simulink model "Trench_Zone"  (R2023b)
settings: Solver=VariableStepAuto  StartTime=0.0  StopTime=10.0  RelTol=1e-3
undefined symbols (not defined in the file or in its folder): Need_Distance_from_Trench, Warning_Threshold_Max_Distance, Warning_Threshold_Min_Distance, Warning_Threshold_Time
settings Model: Creator=Bing  LastModifiedBy=Bing

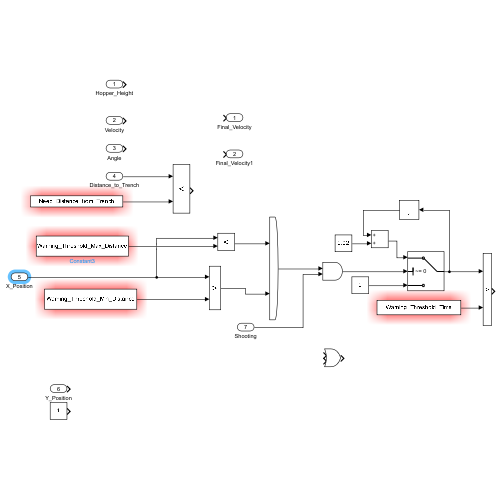
[thumbnail: Simulink's stored preview of the top-level diagram]
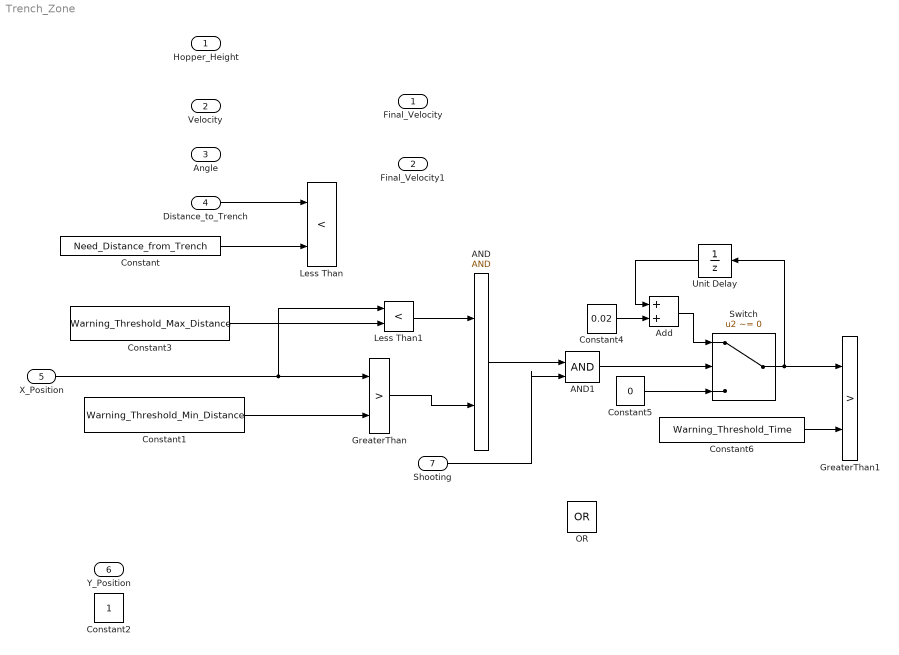
== system Trench_Zone ==
  Hopper_Height : Inport
  Velocity : Inport  Port=2
  Angle : Inport  Port=3
  Distance_to_Trench : Inport  Port=4
  X_Position : Inport  Port=5
  Y_Position : Inport  Port=6
  Shooting : Inport  Port=7
  AND : Logic  IconShape=distinctive  AllPortsSameDT=off  OutDataTypeStr=boolean
  AND1 : Logic  IconShape=distinctive  AllPortsSameDT=off  OutDataTypeStr=boolean
  Add : Sum
  Constant : Constant  Value=Need_Distance_from_Trench
  Constant1 : Constant  Value=Warning_Threshold_Min_Distance
  Constant2 : Constant
  Constant3 : Constant  Value=Warning_Threshold_Max_Distance
  Constant4 : Constant  Value=0.02
  Constant5 : Constant  Value=0
  Constant6 : Constant  Value=Warning_Threshold_Time
  GreaterThan : RelationalOperator  Operator=>  OutDataTypeStr=boolean  RndMeth=Simplest  InputSameDT=off
  GreaterThan1 : RelationalOperator  Operator=>  OutDataTypeStr=boolean  RndMeth=Simplest  InputSameDT=off
  Less Than : RelationalOperator  Operator=<  OutDataTypeStr=boolean  RndMeth=Simplest  InputSameDT=off
  Less Than1 : RelationalOperator  Operator=<  OutDataTypeStr=boolean  RndMeth=Simplest  InputSameDT=off
  OR : Logic  Operator=OR  IconShape=distinctive  AllPortsSameDT=off  OutDataTypeStr=boolean
  Switch : Switch  Criteria=u2 ~= 0  SaturateOnIntegerOverflow=off  InputSameDT=off
  Unit Delay : UnitDelay  SampleTime=-1  HasFrameUpgradeWarning=on
  Final_Velocity : Outport
  Final_Velocity1 : Outport  Port=2
  wires:
  Distance_to_Trench/1 -> Less Than/1
  Constant/1 -> Less Than/2
  X_Position/1 -> Less Than1/1, GreaterThan/1
  Constant1/1 -> GreaterThan/2
  GreaterThan/1 -> AND/2
  Constant3/1 -> Less Than1/2
  Less Than1/1 -> AND/1
  AND/1 -> AND1/1
  Shooting/1 -> AND1/2
  AND1/1 -> Switch/2
  Switch/1 -> GreaterThan1/1, Unit Delay/1
  Add/1 -> Switch/1
  Constant4/1 -> Add/2
  Constant5/1 -> Switch/3
  Unit Delay/1 -> Add/1
  Constant6/1 -> GreaterThan1/2
